simulink library "CurrentReference"  (R2026a)
settings: Solver=VariableStepAuto
undefined symbols (not defined in the file): pmsmCfg, refCfg
libraries: $bdroot x3
settings Model: Creator=24322  LastModifiedBy=24322

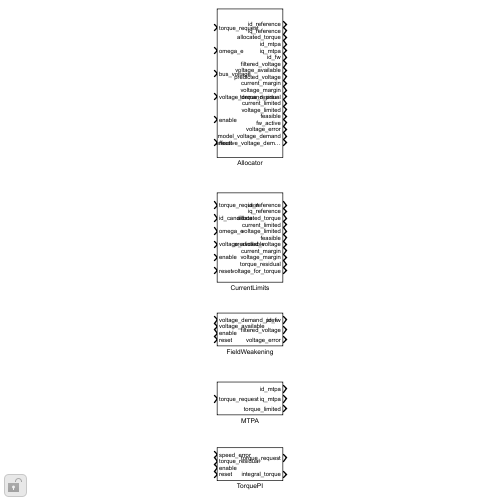
[thumbnail: Simulink's stored preview of the top-level diagram]
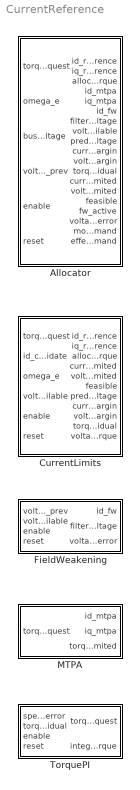
== system CurrentReference ==
  Allocator : Subsystem
  CurrentLimits : Subsystem
  FieldWeakening : Subsystem
  MTPA : Subsystem
  TorquePI : Subsystem

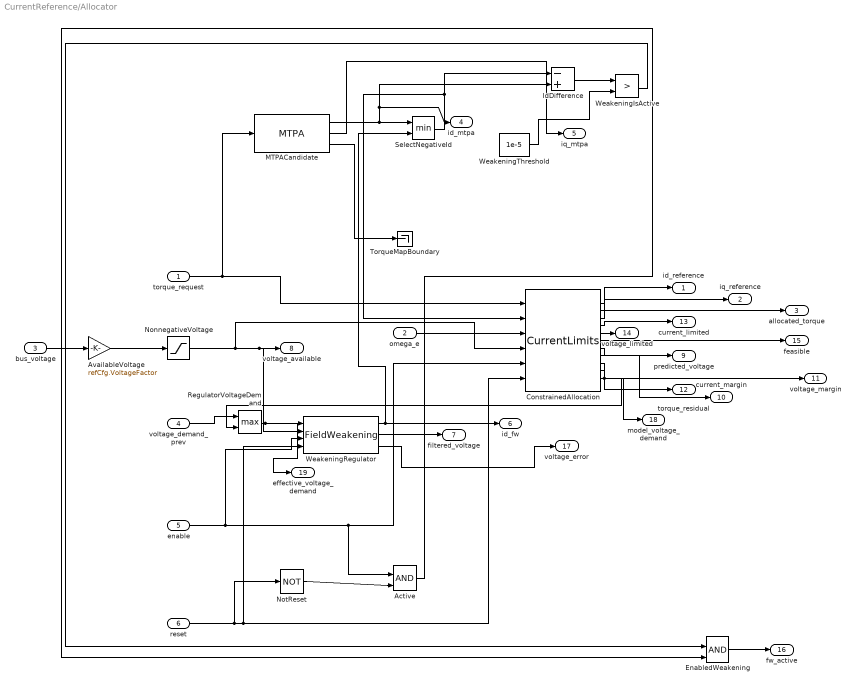
== system CurrentReference/Allocator ==
  torque_request : Inport
  omega_e : Inport  Port=2
  bus_voltage : Inport  Port=3
  voltage_demand_prev : Inport  Port=4
  enable : Inport  Port=5
  reset : Inport  Port=6
  Active : Logic  IconShape=distinctive  AllPortsSameDT=off  OutDataTypeStr=boolean
  AvailableVoltage : Gain  Gain=refCfg.VoltageFactor
  ConstrainedAllocation : $bdroot/CurrentLimits  SystemSampleTime=-1  VariantActivationTime=update diagram  EmptyChoice=off  PassThrough=off  PassThroughVariantControl=(default)  EmptyChoiceVariantControl=(default)  AllowFlexibleInterface=on  Latency=0  AutoFrameSizeCalculation=off
  EnabledWeakening : Logic  IconShape=distinctive  AllPortsSameDT=off  OutDataTypeStr=boolean
  IdDifference : Sum  Inputs=-+
  MTPACandidate : $bdroot/MTPA  SystemSampleTime=-1  VariantActivationTime=update diagram  EmptyChoice=off  PassThrough=off  PassThroughVariantControl=(default)  EmptyChoiceVariantControl=(default)  AllowFlexibleInterface=on  Latency=0  AutoFrameSizeCalculation=off
  NonnegativeVoltage : Saturate  UpperLimit=inf  LowerLimit=0
  NotReset : Logic  Operator=NOT  IconShape=distinctive  AllPortsSameDT=off  OutDataTypeStr=boolean
  RegulatorVoltageDemand : MinMax  Function=max  Inputs=2
  SelectNegativeId : MinMax  Inputs=2
  TorqueMapBoundary : Terminator
  WeakeningIsActive : RelationalOperator  Operator=>  OutDataTypeStr=boolean  RndMeth=Simplest  InputSameDT=off
  WeakeningRegulator : $bdroot/FieldWeakening  SystemSampleTime=-1  VariantActivationTime=update diagram  EmptyChoice=off  PassThrough=off  PassThroughVariantControl=(default)  EmptyChoiceVariantControl=(default)  AllowFlexibleInterface=on  Latency=0  AutoFrameSizeCalculation=off
  WeakeningThreshold : Constant  Value=1e-5
  id_reference : Outport
  iq_reference : Outport  Port=2
  allocated_torque : Outport  Port=3
  id_mtpa : Outport  Port=4
  iq_mtpa : Outport  Port=5
  id_fw : Outport  Port=6
  filtered_voltage : Outport  Port=7
  voltage_available : Outport  Port=8
  predicted_voltage : Outport  Port=9
  current_margin : Outport  Port=10
  voltage_margin : Outport  Port=11
  torque_residual : Outport  Port=12
  current_limited : Outport  Port=13
  voltage_limited : Outport  Port=14
  feasible : Outport  Port=15
  fw_active : Outport  Port=16
  voltage_error : Outport  Port=17
  model_voltage_demand : Outport  Port=18
  effective_voltage_demand : Outport  Port=19
  wires:
  MTPACandidate/2 -> iq_mtpa/1
  NotReset/1 -> Active/2
  MTPACandidate/3 -> TorqueMapBoundary/1
  AvailableVoltage/1 -> NonnegativeVoltage/1
  bus_voltage/1 -> AvailableVoltage/1
  torque_request/1 -> ConstrainedAllocation/1, MTPACandidate/1
  omega_e/1 -> ConstrainedAllocation/3
  NonnegativeVoltage/1 -> WeakeningRegulator/2, voltage_available/1, ConstrainedAllocation/4
  enable/1 -> ConstrainedAllocation/5, Active/1, WeakeningRegulator/3
  reset/1 -> ConstrainedAllocation/6, WeakeningRegulator/4, NotReset/1
  MTPACandidate/1 -> id_mtpa/1, IdDifference/2, SelectNegativeId/1
  WeakeningRegulator/1 -> id_fw/1, SelectNegativeId/2
  SelectNegativeId/1 -> IdDifference/1, ConstrainedAllocation/2
  WeakeningRegulator/3 -> voltage_error/1
  IdDifference/1 -> WeakeningIsActive/1
  WeakeningThreshold/1 -> WeakeningIsActive/2
  WeakeningIsActive/1 -> EnabledWeakening/1
  Active/1 -> EnabledWeakening/2
  ConstrainedAllocation/1 -> id_reference/1
  ConstrainedAllocation/2 -> iq_reference/1
  ConstrainedAllocation/3 -> allocated_torque/1
  WeakeningRegulator/2 -> filtered_voltage/1
  ConstrainedAllocation/7 -> predicted_voltage/1
  ConstrainedAllocation/9 -> voltage_margin/1
  ConstrainedAllocation/10 -> torque_residual/1
  ConstrainedAllocation/4 -> current_limited/1
  ConstrainedAllocation/5 -> voltage_limited/1
  ConstrainedAllocation/6 -> feasible/1
  EnabledWeakening/1 -> fw_active/1
  ConstrainedAllocation/11 -> model_voltage_demand/1, RegulatorVoltageDemand/2
  RegulatorVoltageDemand/1 -> WeakeningRegulator/1, effective_voltage_demand/1
  voltage_demand_prev/1 -> RegulatorVoltageDemand/1
  ConstrainedAllocation/8 -> current_margin/1

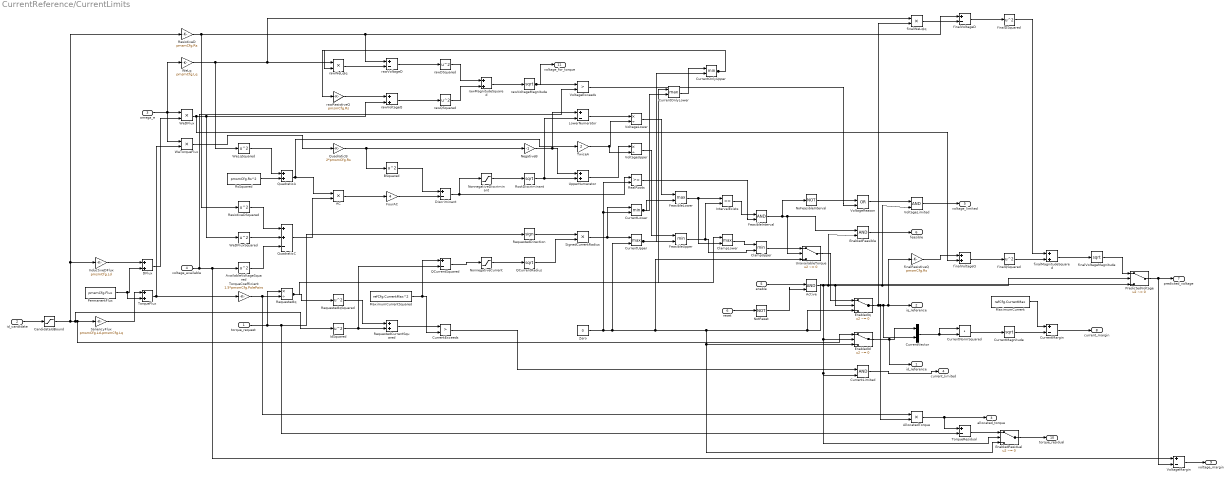
== system CurrentReference/CurrentLimits ==
  torque_request : Inport
  id_candidate : Inport  Port=2
  omega_e : Inport  Port=3
  voltage_available : Inport  Port=4
  enable : Inport  Port=5
  reset : Inport  Port=6
  AC : Product
  Active : Logic  IconShape=distinctive  AllPortsSameDT=off  OutDataTypeStr=boolean
  AllocatedTorque : Product
  AvailableVoltageSquared : Math  Operator=square
  BSquared : Math  Operator=square
  CandidateIdBound : Saturate  UpperLimit=0  LowerLimit=refCfg.IdMin
  ClampLower : MinMax  Function=max  Inputs=2
  ClampUpper : MinMax  Inputs=2
  CurrentExceeds : RelationalOperator  Operator=>  OutDataTypeStr=boolean  RndMeth=Simplest  InputSameDT=off
  CurrentLimited : Logic  IconShape=distinctive  AllPortsSameDT=off  OutDataTypeStr=boolean
  CurrentLower : MinMax  Inputs=2
  CurrentMagnitude : Math  Operator=sqrt
  CurrentMargin : Sum  Inputs=+-
  CurrentNormSquared : DotProduct  OutDataTypeStr=Inherit: Inherit via internal rule
  CurrentOnlyLower : MinMax  Function=max  Inputs=2
  CurrentOnlyUpper : MinMax  Inputs=2
  CurrentUpper : MinMax  Function=max  Inputs=2
  CurrentVector : Mux  Inputs=2
  DFlux : Sum
  Discriminant : Sum  Inputs=+-
  EnabledFeasible : Logic  IconShape=distinctive  AllPortsSameDT=off  OutDataTypeStr=boolean
  EnabledId : Switch  Criteria=u2 ~= 0  SaturateOnIntegerOverflow=off  InputSameDT=off
  EnabledIq : Switch  Criteria=u2 ~= 0  SaturateOnIntegerOverflow=off  InputSameDT=off
  EnabledResidual : Switch  Criteria=u2 ~= 0  SaturateOnIntegerOverflow=off  InputSameDT=off
  FeasibleInterval : Logic  IconShape=distinctive  AllPortsSameDT=off  OutDataTypeStr=boolean
  FeasibleLower : MinMax  Function=max  Inputs=2
  FeasibleUpper : MinMax  Inputs=2
  FourAC : Gain  Gain=4
  IdSquared : Math  Operator=square
  InductiveDFlux : Gain  Gain=pmsmCfg.Ld
  IntervalExists : RelationalOperator  Operator=<=  OutDataTypeStr=boolean  RndMeth=Simplest  InputSameDT=off
  LowerNumerator : Sum  Inputs=+-
  MaximumCurrent : Constant  Value=refCfg.CurrentMax
  MaximumCurrentSquared : Constant  Value=refCfg.CurrentMax^2
  NegativeB : Gain  Gain=-1
  NoFeasibleInterval : Logic  Operator=NOT  IconShape=distinctive  AllPortsSameDT=off  OutDataTypeStr=boolean
  NonnegativeCurrent : Saturate  UpperLimit=inf  LowerLimit=0
  NonnegativeDiscriminant : Saturate  UpperLimit=inf  LowerLimit=0
  NotReset : Logic  Operator=NOT  IconShape=distinctive  AllPortsSameDT=off  OutDataTypeStr=boolean
  PermanentFlux : Constant  Value=pmsmCfg.Flux
  PredictedVoltage : Switch  Criteria=u2 ~= 0  SaturateOnIntegerOverflow=off  InputSameDT=off
  QCurrentRadius : Math  Operator=sqrt
  QCurrentSquared : Sum  Inputs=+-
  QuadraticA : Sum
  QuadraticB : Gain  Gain=2*pmsmCfg.Rs
  QuadraticC : Sum  Inputs=++-
  RealRoots : RelationalOperator  OutDataTypeStr=boolean  RndMeth=Simplest  InputSameDT=off
  RequestedCurrentSquared : Sum
  RequestedDirection : Signum
  RequestedIq : Product  Inputs=*/
  RequestedIqSquared : Math  Operator=square
  ResistiveD : Gain  Gain=pmsmCfg.Rs
  ResistiveDSquared : Math  Operator=square
  RootDiscriminant : Math  Operator=sqrt
  RsSquared : Constant  Value=pmsmCfg.Rs^2
  SaliencyFlux : Gain  Gain=pmsmCfg.Ld-pmsmCfg.Lq
  SignedCurrentRadius : Product
  TorqueCoefficient : Gain  Gain=1.5*pmsmCfg.PolePairs
  TorqueFlux : Sum
  TorqueResidual : Sum  Inputs=+-
  TwiceA : Gain  Gain=2
  UnavailableTorque : Switch  Criteria=u2 ~= 0  SaturateOnIntegerOverflow=off  InputSameDT=off
  UpperNumerator : Sum
  VoltageExceeds : RelationalOperator  Operator=>  OutDataTypeStr=boolean  RndMeth=Simplest  InputSameDT=off
  VoltageLimited : Logic  IconShape=distinctive  AllPortsSameDT=off  OutDataTypeStr=boolean
  VoltageLower : Product  Inputs=*/
  VoltageMargin : Sum  Inputs=+-
  VoltageReason : Logic  Operator=OR  IconShape=distinctive  AllPortsSameDT=off  OutDataTypeStr=boolean
  VoltageUpper : Product  Inputs=*/
  WeDFlux : Product
  WeDFluxSquared : Math  Operator=square
  WeLq : Gain  Gain=pmsmCfg.Lq
  WeLqSquared : Math  Operator=square
  WeTorqueFlux : Product
  Zero : Constant  Value=0
  finalDSquared : Math  Operator=square
  finalMagnitudeSquared : Sum
  finalQSquared : Math  Operator=square
  finalResistiveQ : Gain  Gain=pmsmCfg.Rs
  finalVoltageD : Sum  Inputs=+-
  finalVoltageMagnitude : Math  Operator=sqrt
  finalVoltageQ : Sum
  finalWeLqIq : Product
  rawDSquared : Math  Operator=square
  rawMagnitudeSquared : Sum
  rawQSquared : Math  Operator=square
  rawResistiveQ : Gain  Gain=pmsmCfg.Rs
  rawVoltageD : Sum  Inputs=+-
  rawVoltageMagnitude : Math  Operator=sqrt
  rawVoltageQ : Sum
  rawWeLqIq : Product
  id_reference : Outport
  iq_reference : Outport  Port=2
  allocated_torque : Outport  Port=3
  current_limited : Outport  Port=4
  voltage_limited : Outport  Port=5
  feasible : Outport  Port=6
  predicted_voltage : Outport  Port=7
  current_margin : Outport  Port=8
  voltage_margin : Outport  Port=9
  torque_residual : Outport  Port=10
  voltage_for_torque : Outport  Port=11
  wires:
  EnabledResidual/1 -> torque_residual/1
  VoltageMargin/1 -> voltage_margin/1
  CurrentMargin/1 -> current_margin/1
  EnabledFeasible/1 -> feasible/1
  VoltageLimited/1 -> voltage_limited/1
  CurrentLimited/1 -> current_limited/1
  finalVoltageMagnitude/1 -> PredictedVoltage/1
  VoltageExceeds/1 -> VoltageReason/2
  finalMagnitudeSquared/1 -> finalVoltageMagnitude/1
  finalQSquared/1 -> finalMagnitudeSquared/2
  finalDSquared/1 -> finalMagnitudeSquared/1
  finalVoltageQ/1 -> finalQSquared/1
  finalVoltageD/1 -> finalDSquared/1
  finalResistiveQ/1 -> finalVoltageQ/1
  finalWeLqIq/1 -> finalVoltageD/2
  rawMagnitudeSquared/1 -> rawVoltageMagnitude/1
  rawQSquared/1 -> rawMagnitudeSquared/2
  rawDSquared/1 -> rawMagnitudeSquared/1
  rawVoltageQ/1 -> rawQSquared/1
  rawVoltageD/1 -> rawDSquared/1
  rawResistiveQ/1 -> rawVoltageQ/1
  rawWeLqIq/1 -> rawVoltageD/2
  PredictedVoltage/1 -> VoltageMargin/2, predicted_voltage/1
  CurrentMagnitude/1 -> CurrentMargin/2
  MaximumCurrent/1 -> CurrentMargin/1
  CurrentNormSquared/1 -> CurrentMagnitude/1
  CurrentVector/1 -> CurrentNormSquared/1, CurrentNormSquared/2
  EnabledId/1 -> CurrentVector/1, id_reference/1
  VoltageReason/1 -> VoltageLimited/1
  NoFeasibleInterval/1 -> VoltageReason/1
  CurrentExceeds/1 -> CurrentLimited/1
  RequestedCurrentSquared/1 -> CurrentExceeds/1
  RequestedIqSquared/1 -> RequestedCurrentSquared/1
  TorqueResidual/1 -> EnabledResidual/1
  AllocatedTorque/1 -> TorqueResidual/1, allocated_torque/1
  EnabledIq/1 -> finalResistiveQ/1, iq_reference/1, CurrentVector/2, AllocatedTorque/2, finalWeLqIq/2
  UnavailableTorque/1 -> EnabledIq/1
  Active/1 -> CurrentLimited/2, EnabledResidual/2, EnabledId/2, VoltageLimited/2, PredictedVoltage/2, EnabledIq/2, EnabledFeasible/2
  NotReset/1 -> Active/2
  enable/1 -> Active/1
  reset/1 -> NotReset/1
  FeasibleInterval/1 -> UnavailableTorque/2, EnabledFeasible/1, NoFeasibleInterval/1
  ClampUpper/1 -> UnavailableTorque/1
  ClampLower/1 -> ClampUpper/1
  RealRoots/1 -> FeasibleInterval/2
  IntervalExists/1 -> FeasibleInterval/1
  FeasibleUpper/1 -> IntervalExists/2, ClampUpper/2
  FeasibleLower/1 -> IntervalExists/1, ClampLower/2
  VoltageUpper/1 -> FeasibleUpper/1
  VoltageLower/1 -> FeasibleLower/1
  UpperNumerator/1 -> VoltageUpper/1
  TwiceA/1 -> VoltageLower/2, VoltageUpper/2
  LowerNumerator/1 -> VoltageLower/1
  RootDiscriminant/1 -> LowerNumerator/2, UpperNumerator/2
  NegativeB/1 -> LowerNumerator/1, UpperNumerator/1
  NonnegativeDiscriminant/1 -> RootDiscriminant/1
  Discriminant/1 -> NonnegativeDiscriminant/1, RealRoots/1
  FourAC/1 -> Discriminant/2
  BSquared/1 -> Discriminant/1
  AC/1 -> FourAC/1
  QuadraticC/1 -> AC/2
  QuadraticA/1 -> TwiceA/1, AC/1
  QuadraticB/1 -> NegativeB/1, BSquared/1
  AvailableVoltageSquared/1 -> QuadraticC/3
  WeDFluxSquared/1 -> QuadraticC/2
  ResistiveDSquared/1 -> QuadraticC/1
  voltage_available/1 -> AvailableVoltageSquared/1, VoltageMargin/1, VoltageExceeds/2
  WeDFlux/1 -> WeDFluxSquared/1, rawVoltageQ/2, finalVoltageQ/2
  DFlux/1 -> WeDFlux/2
  InductiveDFlux/1 -> DFlux/1
  ResistiveD/1 -> rawVoltageD/1, finalVoltageD/1, ResistiveDSquared/1
  WeTorqueFlux/1 -> QuadraticB/1
  RsSquared/1 -> QuadraticA/2
  WeLqSquared/1 -> QuadraticA/1
  WeLq/1 -> rawWeLqIq/1, finalWeLqIq/1, WeLqSquared/1
  omega_e/1 -> WeTorqueFlux/1, WeDFlux/1, WeLq/1
  TorqueCoefficient/1 -> RequestedIq/2, AllocatedTorque/1
  TorqueFlux/1 -> TorqueCoefficient/1, WeTorqueFlux/2
  PermanentFlux/1 -> TorqueFlux/2, DFlux/2
  SaliencyFlux/1 -> TorqueFlux/1
  Zero/1 -> EnabledResidual/3, EnabledId/3, PredictedVoltage/3, EnabledIq/3, UnavailableTorque/3, CurrentUpper/2, CurrentLower/2, RealRoots/2
  SignedCurrentRadius/1 -> CurrentLower/1, CurrentUpper/1
  QCurrentRadius/1 -> SignedCurrentRadius/2
  RequestedDirection/1 -> SignedCurrentRadius/1
  torque_request/1 -> TorqueResidual/2, RequestedDirection/1, RequestedIq/1
  NonnegativeCurrent/1 -> QCurrentRadius/1
  QCurrentSquared/1 -> NonnegativeCurrent/1
  IdSquared/1 -> QCurrentSquared/2, RequestedCurrentSquared/2
  MaximumCurrentSquared/1 -> QCurrentSquared/1, CurrentExceeds/2
  CandidateIdBound/1 -> SaliencyFlux/1, EnabledId/1, IdSquared/1, ResistiveD/1, InductiveDFlux/1
  id_candidate/1 -> CandidateIdBound/1
  CurrentOnlyUpper/1 -> rawResistiveQ/1, rawWeLqIq/2
  CurrentOnlyLower/1 -> CurrentOnlyUpper/1
  CurrentLower/1 -> CurrentOnlyLower/2, FeasibleLower/2
  CurrentUpper/1 -> CurrentOnlyUpper/2, FeasibleUpper/2
  RequestedIq/1 -> CurrentOnlyLower/1, RequestedIqSquared/1, ClampLower/1
  rawVoltageMagnitude/1 -> voltage_for_torque/1, VoltageExceeds/1

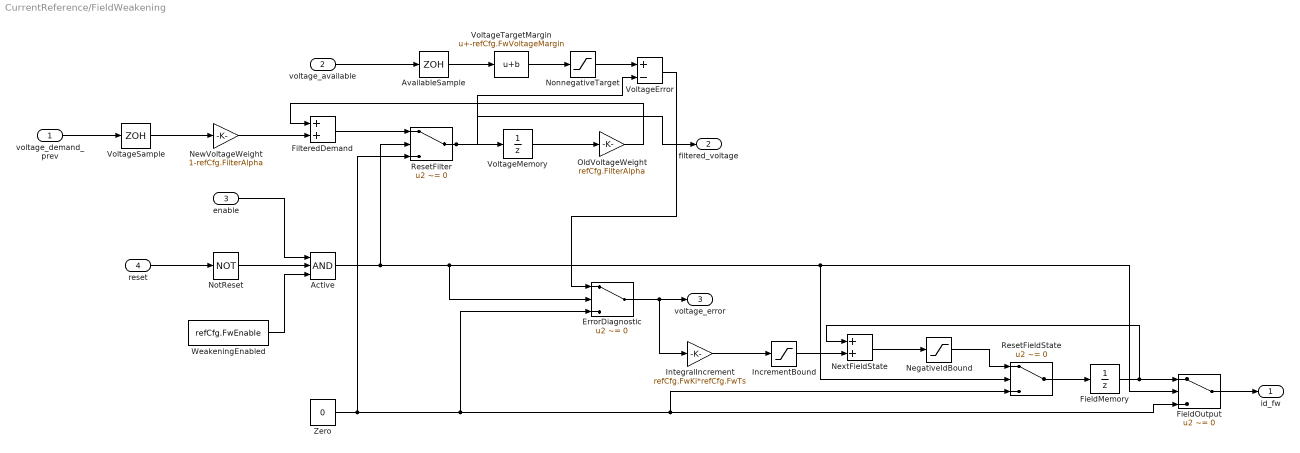
== system CurrentReference/FieldWeakening ==
  voltage_demand_prev : Inport
  voltage_available : Inport  Port=2
  enable : Inport  Port=3
  reset : Inport  Port=4
  Active : Logic  Inputs=3  IconShape=distinctive  AllPortsSameDT=off  OutDataTypeStr=boolean
  AvailableSample : ZeroOrderHold  SampleTime=refCfg.FwTs
  ErrorDiagnostic : Switch  Criteria=u2 ~= 0  SaturateOnIntegerOverflow=off  InputSameDT=off
  FieldMemory : UnitDelay  SampleTime=refCfg.FwTs
  FieldOutput : Switch  Criteria=u2 ~= 0  SaturateOnIntegerOverflow=off  InputSameDT=off
  FilteredDemand : Sum
  IncrementBound : Saturate  UpperLimit=refCfg.IdSlew*refCfg.FwTs  LowerLimit=-refCfg.IdSlew*refCfg.FwTs
  IntegralIncrement : Gain  Gain=refCfg.FwKi*refCfg.FwTs
  NegativeIdBound : Saturate  UpperLimit=0  LowerLimit=refCfg.IdMin
  NewVoltageWeight : Gain  Gain=1-refCfg.FilterAlpha
  NextFieldState : Sum
  NonnegativeTarget : Saturate  UpperLimit=inf  LowerLimit=0
  NotReset : Logic  Operator=NOT  IconShape=distinctive  AllPortsSameDT=off  OutDataTypeStr=boolean
  OldVoltageWeight : Gain  Gain=refCfg.FilterAlpha
  ResetFieldState : Switch  Criteria=u2 ~= 0  SaturateOnIntegerOverflow=off  InputSameDT=off
  ResetFilter : Switch  Criteria=u2 ~= 0  SaturateOnIntegerOverflow=off  InputSameDT=off
  VoltageError : Sum  Inputs=+-
  VoltageMemory : UnitDelay  SampleTime=refCfg.FwTs
  VoltageSample : ZeroOrderHold  SampleTime=refCfg.FwTs
  VoltageTargetMargin : Bias  Bias=-refCfg.FwVoltageMargin  SaturateOnIntegerOverflow=off
  WeakeningEnabled : Constant  Value=refCfg.FwEnable
  Zero : Constant  Value=0
  id_fw : Outport
  filtered_voltage : Outport  Port=2
  voltage_error : Outport  Port=3
  wires:
  FieldOutput/1 -> id_fw/1
  ResetFieldState/1 -> FieldMemory/1
  NegativeIdBound/1 -> ResetFieldState/1
  NextFieldState/1 -> NegativeIdBound/1
  IncrementBound/1 -> NextFieldState/2
  FieldMemory/1 -> NextFieldState/1, FieldOutput/1
  IntegralIncrement/1 -> IncrementBound/1
  ErrorDiagnostic/1 -> IntegralIncrement/1, voltage_error/1
  Zero/1 -> ResetFieldState/3, FieldOutput/3, ErrorDiagnostic/3, ResetFilter/3
  Active/1 -> ResetFieldState/2, FieldOutput/2, ErrorDiagnostic/2, ResetFilter/2
  FilteredDemand/1 -> ResetFilter/1
  WeakeningEnabled/1 -> Active/3
  NotReset/1 -> Active/2
  enable/1 -> Active/1
  reset/1 -> NotReset/1
  NewVoltageWeight/1 -> FilteredDemand/2
  OldVoltageWeight/1 -> FilteredDemand/1
  VoltageMemory/1 -> OldVoltageWeight/1
  VoltageSample/1 -> NewVoltageWeight/1
  voltage_available/1 -> AvailableSample/1
  voltage_demand_prev/1 -> VoltageSample/1
  NonnegativeTarget/1 -> VoltageError/1
  VoltageTargetMargin/1 -> NonnegativeTarget/1
  ResetFilter/1 -> filtered_voltage/1, VoltageMemory/1, VoltageError/2
  AvailableSample/1 -> VoltageTargetMargin/1
  VoltageError/1 -> ErrorDiagnostic/1

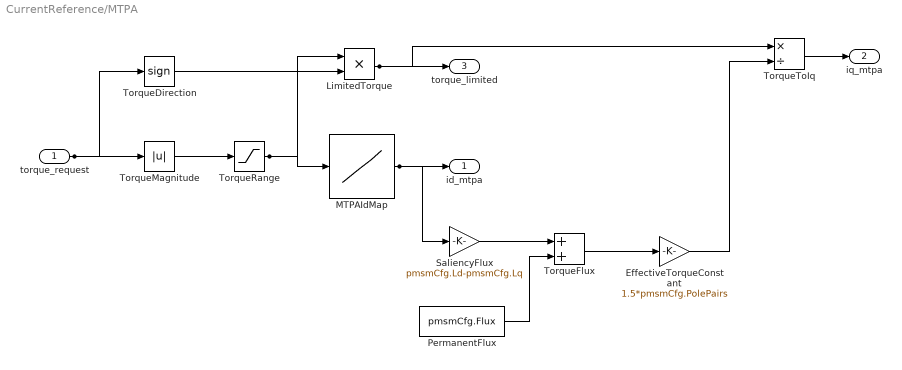
== system CurrentReference/MTPA ==
  torque_request : Inport
  EffectiveTorqueConstant : Gain  Gain=1.5*pmsmCfg.PolePairs
  LimitedTorque : Product
  MTPAIdMap : Lookup_n-D  NumberOfTableDimensions=1  BreakpointsForDimension1=refCfg.TorqueGrid  Table=refCfg.IdTable  ExtrapMethod=Clip  InternalRulePriority=Speed  RndMeth=Simplest
  PermanentFlux : Constant  Value=pmsmCfg.Flux
  SaliencyFlux : Gain  Gain=pmsmCfg.Ld-pmsmCfg.Lq
  TorqueDirection : Signum
  TorqueFlux : Sum
  TorqueMagnitude : Abs  SaturateOnIntegerOverflow=off
  TorqueRange : Saturate  UpperLimit=refCfg.MaxTorque  LowerLimit=0
  TorqueToIq : Product  Inputs=*/
  id_mtpa : Outport
  iq_mtpa : Outport  Port=2
  torque_limited : Outport  Port=3
  wires:
  TorqueToIq/1 -> iq_mtpa/1
  EffectiveTorqueConstant/1 -> TorqueToIq/2
  LimitedTorque/1 -> TorqueToIq/1, torque_limited/1
  TorqueFlux/1 -> EffectiveTorqueConstant/1
  PermanentFlux/1 -> TorqueFlux/2
  SaliencyFlux/1 -> TorqueFlux/1
  MTPAIdMap/1 -> SaliencyFlux/1, id_mtpa/1
  TorqueDirection/1 -> LimitedTorque/2
  TorqueRange/1 -> LimitedTorque/1, MTPAIdMap/1
  TorqueMagnitude/1 -> TorqueRange/1
  torque_request/1 -> TorqueMagnitude/1, TorqueDirection/1

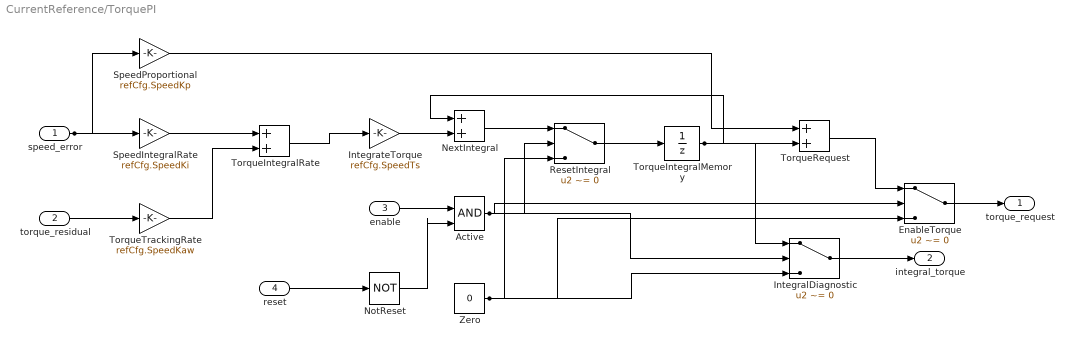
== system CurrentReference/TorquePI ==
  speed_error : Inport
  torque_residual : Inport  Port=2
  enable : Inport  Port=3
  reset : Inport  Port=4
  Active : Logic  IconShape=distinctive  AllPortsSameDT=off  OutDataTypeStr=boolean
  EnableTorque : Switch  Criteria=u2 ~= 0  SaturateOnIntegerOverflow=off  InputSameDT=off
  IntegralDiagnostic : Switch  Criteria=u2 ~= 0  SaturateOnIntegerOverflow=off  InputSameDT=off
  IntegrateTorque : Gain  Gain=refCfg.SpeedTs
  NextIntegral : Sum
  NotReset : Logic  Operator=NOT  IconShape=distinctive  AllPortsSameDT=off  OutDataTypeStr=boolean
  ResetIntegral : Switch  Criteria=u2 ~= 0  SaturateOnIntegerOverflow=off  InputSameDT=off
  SpeedIntegralRate : Gain  Gain=refCfg.SpeedKi
  SpeedProportional : Gain  Gain=refCfg.SpeedKp
  TorqueIntegralMemory : UnitDelay  SampleTime=refCfg.SpeedTs
  TorqueIntegralRate : Sum
  TorqueRequest : Sum
  TorqueTrackingRate : Gain  Gain=refCfg.SpeedKaw
  Zero : Constant  Value=0
  torque_request : Outport
  integral_torque : Outport  Port=2
  wires:
  IntegralDiagnostic/1 -> integral_torque/1
  EnableTorque/1 -> torque_request/1
  TorqueRequest/1 -> EnableTorque/1
  ResetIntegral/1 -> TorqueIntegralMemory/1
  Zero/1 -> ResetIntegral/3, EnableTorque/3, IntegralDiagnostic/3
  Active/1 -> ResetIntegral/2, EnableTorque/2, IntegralDiagnostic/2
  NextIntegral/1 -> ResetIntegral/1
  NotReset/1 -> Active/2
  enable/1 -> Active/1
  reset/1 -> NotReset/1
  SpeedProportional/1 -> TorqueRequest/1
  IntegrateTorque/1 -> NextIntegral/2
  TorqueIntegralMemory/1 -> IntegralDiagnostic/1, NextIntegral/1, TorqueRequest/2
  TorqueIntegralRate/1 -> IntegrateTorque/1
  TorqueTrackingRate/1 -> TorqueIntegralRate/2
  SpeedIntegralRate/1 -> TorqueIntegralRate/1
  torque_residual/1 -> TorqueTrackingRate/1
  speed_error/1 -> SpeedProportional/1, SpeedIntegralRate/1
